simulink model "PrmM_CustomerLimits"  (R2018b)
settings: Solver=FixedStepDiscrete  StartTime=0.0  StopTime=20  RelTol=1e-3  EnableMultiTasking=on
undefined symbols (not defined in the file): CS_PrmM_nHSpdBd_XDF32, CS_PrmM_nLwrSpdBd_XDF32, CS_PrmM_uDcMaxVoltMode_XDF32, CS_PrmM_uDcMinVoltMode_XDF32
libraries: CalibrationLib x1
(part 2 of 2)

== stateflow chart PrmM_CustomerLimits/Test Sequence ==
  settings: updateMethod=DISCRETE  sampleTime=0.001  stateMachineType=SIMPLIFIED_MACHINE
  state Run
    %% Initialize data outputs.
    DrvM_Inp_sState = AD_DrvM_tSTATEIDX_E.CS_DrvM_STATE_Idle;
    ModeReqInt_Inp_sIntReqMode = AD_DrvM_tSTATEIDX_E.CS_DrvM_STATE_Idle;
    VoltLimExt_Inp_uReqdMinBattU = single(0);
    TqReqLim_Inp_mTqMax = single(0);
    VoltLimExt_Inp_uReqdMaxBattU = single(0);
    PwrLimExt_Inp_pPwrMinLim = single(0);
    PwrLimExt_Inp_pPwrMaxLim = single(0);
    TqDesGrdtExt_Inp_TqDesGrdtExt = single(0);
    Rotp_Inp_nSpdMecl = single(0);
    CurrLimExt_Inp_iReqdMinBattI = single(0);
    ExtTarTqReq_Inp_mReqTqEM = single(0);
    TqLimExt_Inp_mTqLimMin = single(0);
    CurrLimExt_Inp_iReqdMaxBattI = single(0);
    TqLimExt_Inp_mTqLimMax = single(0);
    ExtTarTqReq_Inp_nReqdSpdEM = single(0);
    ExtTarTqReq_Inp_uReqUEM = single(0);
    TqReqLim_Inp_mTqMin = single(0);
    ActTq_Inp_mDragTq = single(0);
    IDcLim_Inp_IDcLimMinInt=single(-290);
    IDcLim_Inp_IDcLimMaxInt=single(360);
    SplyU48_uU48=single(48);
    ElmTqLim_mTqMin=single(-70);
  state TorqueLimits
    state SpeedMode
      DrvM_Inp_sState = AD_DrvM_tSTATEIDX_E.CS_DrvM_STATE_Spd;
      state ExternalLimitsAreTheStrictest
        TqLimExt_Inp_mTqLimMax=single(20);
        TqLimExt_Inp_mTqLimMin=single(-20);
        TqReqLim_Inp_mTqMax=single(65);
        TqReqLim_Inp_mTqMin=single(-60);
        state wait
        state verfiy
          verify(abs(TqLimTarTqCtrl_Outp_mTqLimMax-TqLimExt_Inp_mTqLimMax)<Tolerance)
          verify(abs(TqLimTarTqCtrl_Outp_mTqLimMin-TqLimExt_Inp_mTqLimMin)<Tolerance)
          verify(abs(PwrLimExtCust_Outp_pPwrMaxLim-PwrLimExt_Inp_pPwrMaxLim)<Tolerance)
          verify(abs(PwrLimExtCust_Outp_pPwrMinLim-PwrLimExt_Inp_pPwrMinLim)<Tolerance)
        (default) -> TorqueLimits.SpeedMode.ExternalLimitsAreTheStrictest.wait
        TorqueLimits.SpeedMode.ExternalLimitsAreTheStrictest.wait -> TorqueLimits.SpeedMode.ExternalLimitsAreTheStrictest.verfiy : [after(0.1,sec)
            | ]
      state DeratingLimitsAreTheStrictest
        TqLimExt_Inp_mTqLimMax=single(65);
        TqLimExt_Inp_mTqLimMin=single(-65);
        TqReqLim_Inp_mTqMax=single(20);
        TqReqLim_Inp_mTqMin=single(-20);
        state wait
        state verfiy
          verify(abs(TqLimTarTqCtrl_Outp_mTqLimMax-TqReqLim_Inp_mTqMax)<Tolerance)
          verify(abs(TqLimTarTqCtrl_Outp_mTqLimMin-TqReqLim_Inp_mTqMin)<Tolerance)
          verify(abs(PwrLimExtCust_Outp_pPwrMaxLim-PwrLimExt_Inp_pPwrMaxLim)<Tolerance)
          verify(abs(PwrLimExtCust_Outp_pPwrMinLim-PwrLimExt_Inp_pPwrMinLim)<Tolerance)
        (default) -> TorqueLimits.SpeedMode.DeratingLimitsAreTheStrictest.wait
        TorqueLimits.SpeedMode.DeratingLimitsAreTheStrictest.wait -> TorqueLimits.SpeedMode.DeratingLimitsAreTheStrictest.verfiy : [after(0.1,sec)
            | ]
      state ExtLimitsAboveIntLimits
        TqLimExt_Inp_mTqLimMax=single(65);
        TqLimExt_Inp_mTqLimMin=single(50);
        TqReqLim_Inp_mTqMax=single(20);
        TqReqLim_Inp_mTqMin=single(-65);
        state wait
        state verfiy
          verify(abs(TqLimTarTqCtrl_Outp_mTqLimMax-TqReqLim_Inp_mTqMax)<Tolerance)
          verify(abs(TqLimTarTqCtrl_Outp_mTqLimMin-TqReqLim_Inp_mTqMin)<Tolerance)
          verify(abs(PwrLimExtCust_Outp_pPwrMaxLim-PwrLimExt_Inp_pPwrMaxLim)<Tolerance)
          verify(abs(PwrLimExtCust_Outp_pPwrMinLim-PwrLimExt_Inp_pPwrMinLim)<Tolerance)
        (default) -> TorqueLimits.SpeedMode.ExtLimitsAboveIntLimits.wait
        TorqueLimits.SpeedMode.ExtLimitsAboveIntLimits.wait -> TorqueLimits.SpeedMode.ExtLimitsAboveIntLimits.verfiy : [after(0.1,sec)
            | ]
      state ExtLimitsBelowIntLimits
        TqLimExt_Inp_mTqLimMax=single(-20);
        TqLimExt_Inp_mTqLimMin=single(-65);
        TqReqLim_Inp_mTqMax=single(65);
        TqReqLim_Inp_mTqMin=single(20);
        state wait
        state verfiy
          verify(abs(TqLimTarTqCtrl_Outp_mTqLimMax-TqReqLim_Inp_mTqMax)<Tolerance)
          verify(abs(TqLimTarTqCtrl_Outp_mTqLimMin-TqReqLim_Inp_mTqMin)<Tolerance)
          verify(abs(PwrLimExtCust_Outp_pPwrMaxLim-PwrLimExt_Inp_pPwrMaxLim)<Tolerance)
          verify(abs(PwrLimExtCust_Outp_pPwrMinLim-PwrLimExt_Inp_pPwrMinLim)<Tolerance)
        (default) -> TorqueLimits.SpeedMode.ExtLimitsBelowIntLimits.wait
        TorqueLimits.SpeedMode.ExtLimitsBelowIntLimits.wait -> TorqueLimits.SpeedMode.ExtLimitsBelowIntLimits.verfiy : [after(0.1,sec)
            | ]
      state InvalidExternalTorqueLimits
        TqLimExt_Inp_mTqLimMax=single(-20);
        TqLimExt_Inp_mTqLimMin=single(20);
        TqReqLim_Inp_mTqMax=single(20);
        TqReqLim_Inp_mTqMin=single(-20);
        state wait
        state verfiy
          verify(abs(TqLimTarTqCtrl_Outp_mTqLimMax-TqReqLim_Inp_mTqMax)<Tolerance)
          verify(abs(TqLimTarTqCtrl_Outp_mTqLimMin-TqReqLim_Inp_mTqMin)<Tolerance)
          verify(abs(PwrLimExtCust_Outp_pPwrMaxLim-PwrLimExt_Inp_pPwrMaxLim)<Tolerance)
          verify(abs(PwrLimExtCust_Outp_pPwrMinLim-PwrLimExt_Inp_pPwrMinLim)<Tolerance)
        (default) -> TorqueLimits.SpeedMode.InvalidExternalTorqueLimits.wait
        TorqueLimits.SpeedMode.InvalidExternalTorqueLimits.wait -> TorqueLimits.SpeedMode.InvalidExternalTorqueLimits.verfiy : [after(0.1,sec)
            | ]
      state InvalidInternalTorqueLimits
        TqLimExt_Inp_mTqLimMax=single(-20);
        TqLimExt_Inp_mTqLimMin=single(20);
        TqReqLim_Inp_mTqMax=single(-20);
        TqReqLim_Inp_mTqMin=single(20);
        state wait
        state verfiy
          verify(abs(TqLimTarTqCtrl_Outp_mTqLimMax-TqReqLim_Inp_mTqMin)<Tolerance)
          verify(abs(TqLimTarTqCtrl_Outp_mTqLimMin-TqReqLim_Inp_mTqMax)<Tolerance)
          verify(abs(PwrLimExtCust_Outp_pPwrMaxLim-PwrLimExt_Inp_pPwrMaxLim)<Tolerance)
          verify(abs(PwrLimExtCust_Outp_pPwrMinLim-PwrLimExt_Inp_pPwrMinLim)<Tolerance)
        (default) -> TorqueLimits.SpeedMode.InvalidInternalTorqueLimits.wait
        TorqueLimits.SpeedMode.InvalidInternalTorqueLimits.wait -> TorqueLimits.SpeedMode.InvalidInternalTorqueLimits.verfiy : [after(0.1,sec)
            | ]
      (default) -> TorqueLimits.SpeedMode.ExternalLimitsAreTheStrictest
      TorqueLimits.SpeedMode.ExternalLimitsAreTheStrictest -> TorqueLimits.SpeedMode.DeratingLimitsAreTheStrictest : [after(0.5,sec)
          | ]
      TorqueLimits.SpeedMode.DeratingLimitsAreTheStrictest -> TorqueLimits.SpeedMode.ExtLimitsAboveIntLimits : [after(0.5,sec)
          | ]
      TorqueLimits.SpeedMode.ExtLimitsAboveIntLimits -> TorqueLimits.SpeedMode.ExtLimitsBelowIntLimits : [after(0.5,sec)
          | ]
      TorqueLimits.SpeedMode.ExtLimitsBelowIntLimits -> InvalidExternalTorqueLimits : [after(0.5,sec)
          | ]
      InvalidExternalTorqueLimits -> InvalidInternalTorqueLimits : [after(0.5,sec)
          | ]
    state TorqueMode
      DrvM_Inp_sState = AD_DrvM_tSTATEIDX_E.CS_DrvM_STATE_Tq;
      TqLimExt_Inp_mTqLimMax=single(65);
      TqLimExt_Inp_mTqLimMin=single(-65);
      TqReqLim_Inp_mTqMax=single(20);
      TqReqLim_Inp_mTqMin=single(-20);
      state wait
      state verfiy
        verify(abs(TqLimTarTqCtrl_Outp_mTqLimMax-TqLimExt_Inp_mTqLimMax)<Tolerance)
        verify(abs(TqLimTarTqCtrl_Outp_mTqLimMin-TqLimExt_Inp_mTqLimMin)<Tolerance)
        verify(abs(PwrLimExtCust_Outp_pPwrMaxLim-PwrLimExt_Inp_pPwrMaxLim)<Tolerance)
        verify(abs(PwrLimExtCust_Outp_pPwrMinLim-PwrLimExt_Inp_pPwrMinLim)<Tolerance)
      (default) -> TorqueLimits.TorqueMode.wait
      TorqueLimits.TorqueMode.wait -> TorqueLimits.TorqueMode.verfiy : [after(0.1,sec)
          | ]
    state VoltageMode
      DrvM_Inp_sState = AD_DrvM_tSTATEIDX_E.CS_DrvM_STATE_Volt;
      state MaximumTorqueHigherThanDragTorque
        TqLimExt_Inp_mTqLimMax=single(65);
        TqLimExt_Inp_mTqLimMin=single(-65);
        TqReqLim_Inp_mTqMax=single(20);
        TqReqLim_Inp_mTqMin=single(-20);
        ActTq_Inp_mDragTq=single(0.3);
        ElmTqLim_mTqMin=single(-20);
        state wait
        state verfiy
          verify(abs(TqLimTarTqCtrl_Outp_mTqLimMax+ActTq_Inp_mDragTq)<Tolerance)
          verify(abs(TqLimTarTqCtrl_Outp_mTqLimMin+ActTq_Inp_mDragTq)<Tolerance)
          verify(abs(PwrLimExtCust_Outp_pPwrMaxLim-PwrLimExt_Inp_pPwrMaxLim)<Tolerance)
          verify(abs(PwrLimExtCust_Outp_pPwrMinLim-PwrLimExt_Inp_pPwrMinLim)<Tolerance)
        (default) -> TorqueLimits.VoltageMode.MaximumTorqueHigherThanDragTorque.wait
        TorqueLimits.VoltageMode.MaximumTorqueHigherThanDragTorque.wait -> TorqueLimits.VoltageMode.MaximumTorqueHigherThanDragTorque.verfiy : [after(0.1,sec)
            | ]
      state SpeedHigherThanHSpdBd
        %TqReqLim_Inp_mTqMax=single(0);
        Rotp_Inp_nSpdMecl=single(0.99+CS_PrmM_nHSpdBd_XDF32);
        state wait
        state verfiy
          verify(abs(TqLimTarTqCtrl_Outp_mTqLimMax+ActTq_Inp_mDragTq)<Tolerance)
          verify(abs(TqLimTarTqCtrl_Outp_mTqLimMin-ElmTqLim_mTqMin)<Tolerance)
          verify(abs(PwrLimExtCust_Outp_pPwrMaxLim-PwrLimExt_Inp_pPwrMaxLim)<Tolerance)
          verify(abs(PwrLimExtCust_Outp_pPwrMinLim-PwrLimExt_Inp_pPwrMinLim)<Tolerance)
        (default) -> TorqueLimits.VoltageMode.SpeedHigherThanHSpdBd.wait
        TorqueLimits.VoltageMode.SpeedHigherThanHSpdBd.wait -> TorqueLimits.VoltageMode.SpeedHigherThanHSpdBd.verfiy : [after(0.1,sec)
            | ]
      (default) -> TorqueLimits.VoltageMode.MaximumTorqueHigherThanDragTorque
      TorqueLimits.VoltageMode.MaximumTorqueHigherThanDragTorque -> SpeedHigherThanHSpdBd : [after(0.5,sec)
          | ]
    state CommuincationlossMode
      DrvM_Inp_sState = AD_DrvM_tSTATEIDX_E.CS_DrvM_STATE_ComLoss
      state MaximumTorqueHigherThanDragTorque
        TqLimExt_Inp_mTqLimMax=single(65);
        TqLimExt_Inp_mTqLimMin=single(-65);
        TqReqLim_Inp_mTqMax=single(20);
        TqReqLim_Inp_mTqMin=single(-20);
        Rotp_Inp_nSpdMecl=single(-500);
        ActTq_Inp_mDragTq=single(-0.3);
        state wait
        state verfiy
          verify(abs(TqLimTarTqCtrl_Outp_mTqLimMax+ActTq_Inp_mDragTq)<Tolerance)
          verify(abs(TqLimTarTqCtrl_Outp_mTqLimMin+ActTq_Inp_mDragTq)<Tolerance)
          verify(abs(PwrLimExtCust_Outp_pPwrMaxLim-PwrLimExt_Inp_pPwrMaxLim)<Tolerance)
          verify(abs(PwrLimExtCust_Outp_pPwrMinLim-PwrLimExt_Inp_pPwrMinLim)<Tolerance)
        (default) -> TorqueLimits.CommuincationlossMode.MaximumTorqueHigherThanDragTorque.wait
        TorqueLimits.CommuincationlossMode.MaximumTorqueHigherThanDragTorque.wait -> TorqueLimits.CommuincationlossMode.MaximumTorqueHigherThanDragTorque.verfiy : [after(0.1,sec)
            | ]
      state SpeedBtwHSpdBdAndLwrSpdBd
        %TqReqLim_Inp_mTqMax=single(0);
        Rotp_Inp_nSpdMecl=CS_PrmM_nLwrSpdBd_XDF32+single(50);
        ActTq_Inp_mDragTq=single(0.3);
        TqMinInterpol=(ElmTqLim_mTqMin+ActTq_Inp_mDragTq)*(Rotp_Inp_nSpdMecl-CS_PrmM_nLwrSpdBd_XDF32)/...
        (CS_PrmM_nHSpdBd_XDF32-CS_PrmM_nLwrSpdBd_XDF32)-ActTq_Inp_mDragTq;
        state wait
        state verfiy
          verify(abs(TqLimTarTqCtrl_Outp_mTqLimMax+ActTq_Inp_mDragTq)<Tolerance)
          verify(abs(TqLimTarTqCtrl_Outp_mTqLimMin-TqMinInterpol)<Tolerance)
          verify(abs(PwrLimExtCust_Outp_pPwrMaxLim-PwrLimExt_Inp_pPwrMaxLim)<Tolerance)
          verify(abs(PwrLimExtCust_Outp_pPwrMinLim-PwrLimExt_Inp_pPwrMinLim)<Tolerance)
        (default) -> TorqueLimits.CommuincationlossMode.SpeedBtwHSpdBdAndLwrSpdBd.wait
        TorqueLimits.CommuincationlossMode.SpeedBtwHSpdBdAndLwrSpdBd.wait -> TorqueLimits.CommuincationlossMode.SpeedBtwHSpdBdAndLwrSpdBd.verfiy : [after(0.1,sec)
            | ]
      (default) -> TorqueLimits.CommuincationlossMode.MaximumTorqueHigherThanDragTorque
      TorqueLimits.CommuincationlossMode.MaximumTorqueHigherThanDragTorque -> SpeedBtwHSpdBdAndLwrSpdBd : [after(0.5,sec)
          | ]
    state BatteryDisconnectedMode
      DrvM_Inp_sState = AD_DrvM_tSTATEIDX_E.CS_DrvM_STATE_BattDiscnctd;
      state MaximumTorqueHigherThanDargTorque
        TqLimExt_Inp_mTqLimMax=single(65);
        TqLimExt_Inp_mTqLimMin=single(-65);
        TqReqLim_Inp_mTqMax=single(20);
        TqReqLim_Inp_mTqMin=single(-20);
        ActTq_Inp_mDragTq=single(0.3);
        state wait
        state verfiy
          verify(abs(TqLimTarTqCtrl_Outp_mTqLimMax+ActTq_Inp_mDragTq)<Tolerance)
          verify(abs(TqLimTarTqCtrl_Outp_mTqLimMin-TqReqLim_Inp_mTqMin)<Tolerance)
          verify(abs(PwrLimExtCust_Outp_pPwrMaxLim-PwrLimExt_Inp_pPwrMaxLim)<Tolerance)
          verify(abs(PwrLimExtCust_Outp_pPwrMinLim-PwrLimExt_Inp_pPwrMinLim)<Tolerance)
        (default) -> TorqueLimits.BatteryDisconnectedMode.MaximumTorqueHigherThanDargTorque.wait
        TorqueLimits.BatteryDisconnectedMode.MaximumTorqueHigherThanDargTorque.wait -> TorqueLimits.BatteryDisconnectedMode.MaximumTorqueHigherThanDargTorque.verfiy : [after(0.1,sec)
            | ]
      state MaximumTorqueLowerThanDargTorque
        TqLimExt_Inp_mTqLimMax=single(0);
        ActTq_Inp_mDragTq=single(-0.3);
        Rotp_Inp_nSpdMecl=single(-500);
        state wait
        state verfiy
          verify(abs(TqLimTarTqCtrl_Outp_mTqLimMax-TqLimExt_Inp_mTqLimMax)<Tolerance)
          verify(abs(TqLimTarTqCtrl_Outp_mTqLimMin-TqReqLim_Inp_mTqMin)<Tolerance)
          verify(abs(PwrLimExtCust_Outp_pPwrMaxLim-PwrLimExt_Inp_pPwrMaxLim)<Tolerance)
          verify(abs(PwrLimExtCust_Outp_pPwrMinLim-PwrLimExt_Inp_pPwrMinLim)<Tolerance)
        (default) -> TorqueLimits.BatteryDisconnectedMode.MaximumTorqueLowerThanDargTorque.wait
        TorqueLimits.BatteryDisconnectedMode.MaximumTorqueLowerThanDargTorque.wait -> TorqueLimits.BatteryDisconnectedMode.MaximumTorqueLowerThanDargTorque.verfiy : [after(0.1,sec)
            | ]
      (default) -> MaximumTorqueHigherThanDargTorque
      MaximumTorqueHigherThanDargTorque -> MaximumTorqueLowerThanDargTorque : [after(0.5,sec)
          | ]
    (default) -> SpeedMode
    SpeedMode -> TorqueMode : [after(3.5,sec)
        | ]
    TorqueMode -> VoltageMode : [after(0.5,sec)
        | ]
    VoltageMode -> CommuincationlossMode : [after(1,sec)
        | ]
    CommuincationlossMode -> BatteryDisconnectedMode : [after(1,sec)
        | ]
  state TorqueGrandient
    state InternalLimitsAreSelected
      state wait
      state verfiy
        verify(abs(PrmM_Outp_mMaxTqGrdtInt-single(1000))<Tolerance)
        verify(abs(PwrLimExtCust_Outp_pPwrMaxLim-PwrLimExt_Inp_pPwrMaxLim)<Tolerance)
        verify(abs(PwrLimExtCust_Outp_pPwrMinLim-PwrLimExt_Inp_pPwrMinLim)<Tolerance)
      (default) -> TorqueGrandient.InternalLimitsAreSelected.wait
      TorqueGrandient.InternalLimitsAreSelected.wait -> TorqueGrandient.InternalLimitsAreSelected.verfiy : [(CS_PrmM_fTqGrdSelect_XDB==true)&&after(0.1,sec)
          | ]
    state ExternalLimitsAreSelected
      state ExternalTorqueGrandientIsHigherThan2000Nm
        TqDesGrdtExt_Inp_TqDesGrdtExt = single(2500);
        state wait
        state verfiy
          verify(abs(PrmM_Outp_mMaxTqGrdtInt-single(2000))<Tolerance)
          verify(abs(PwrLimExtCust_Outp_pPwrMaxLim-PwrLimExt_Inp_pPwrMaxLim)<Tolerance)
          verify(abs(PwrLimExtCust_Outp_pPwrMinLim-PwrLimExt_Inp_pPwrMinLim)<Tolerance)
        (default) -> TorqueGrandient.ExternalLimitsAreSelected.ExternalTorqueGrandientIsHigherThan2000Nm.wait
        TorqueGrandient.ExternalLimitsAreSelected.ExternalTorqueGrandientIsHigherThan2000Nm.wait -> TorqueGrandient.ExternalLimitsAreSelected.ExternalTorqueGrandientIsHigherThan2000Nm.verfiy : [after(0.1,sec)
            | ]
      state ExternalTorqueGrandientIsLowerThan2000Nm
        TqDesGrdtExt_Inp_TqDesGrdtExt = single(1500);
        state wait
        state verfiy
          verify(abs(PrmM_Outp_mMaxTqGrdtInt-TqDesGrdtExt_Inp_TqDesGrdtExt)<Tolerance)
          verify(abs(PwrLimExtCust_Outp_pPwrMaxLim-PwrLimExt_Inp_pPwrMaxLim)<Tolerance)
          verify(abs(PwrLimExtCust_Outp_pPwrMinLim-PwrLimExt_Inp_pPwrMinLim)<Tolerance)
        (default) -> TorqueGrandient.ExternalLimitsAreSelected.ExternalTorqueGrandientIsLowerThan2000Nm.wait
        TorqueGrandient.ExternalLimitsAreSelected.ExternalTorqueGrandientIsLowerThan2000Nm.wait -> TorqueGrandient.ExternalLimitsAreSelected.ExternalTorqueGrandientIsLowerThan2000Nm.verfiy : [after(0.1,sec)
            | ]
      state ExternalTorqueGrandientIs0Nm
        TqDesGrdtExt_Inp_TqDesGrdtExt = single(0);
        state wait
        state verfiy
          verify(abs(PrmM_Outp_mMaxTqGrdtInt-single(1000))<Tolerance)
          verify(abs(PwrLimExtCust_Outp_pPwrMaxLim-PwrLimExt_Inp_pPwrMaxLim)<Tolerance)
          verify(abs(PwrLimExtCust_Outp_pPwrMinLim-PwrLimExt_Inp_pPwrMinLim)<Tolerance)
        (default) -> TorqueGrandient.ExternalLimitsAreSelected.ExternalTorqueGrandientIs0Nm.wait
        TorqueGrandient.ExternalLimitsAreSelected.ExternalTorqueGrandientIs0Nm.wait -> TorqueGrandient.ExternalLimitsAreSelected.ExternalTorqueGrandientIs0Nm.verfiy : [after(0.1,sec)
            | ]
      (default) -> ExternalTorqueGrandientIsHigherThan2000Nm
      ExternalTorqueGrandientIsHigherThan2000Nm -> ExternalTorqueGrandientIsLowerThan2000Nm : [after(0.5,sec)
          | ]
      ExternalTorqueGrandientIsLowerThan2000Nm -> ExternalTorqueGrandientIs0Nm : [after(0.5,sec)
          | ]
    (default) -> InternalLimitsAreSelected
    InternalLimitsAreSelected -> ExternalLimitsAreSelected : [CS_PrmM_fTqGrdSelect_XDB==false
        | ]
  state VoltageLimits
    DrvM_Inp_sState = AD_DrvM_tSTATEIDX_E.CS_DrvM_STATE_Volt;
    state ExternalLimitsAreTheStrictest
      if CS_PrmM_fTqGrdSelect_XDB
      VoltLimExt_Inp_uReqdMaxBattU=single(CS_PrmM_uDcMaxVoltMode_XDF32-5);
      VoltLimExt_Inp_uReqdMinBattU=single(CS_PrmM_uDcMinVoltMode_XDF32+5);
      else
      VoltLimExt_Inp_uReqdMaxBattU=single(CS_PrmM_uDcMinVoltMode_XDF32-5);
      VoltLimExt_Inp_uReqdMinBattU=single(CS_PrmM_uDcMaxVoltMode_XDF32+5);
      end
      state wait
      state verfiy
        verify(abs(VoltLimExtCust_Outp_uReqdMaxBattU-VoltLimExt_Inp_uReqdMaxBattU)<Tolerance)
        verify(abs(VoltLimExtCust_Outp_uReqdMinBattU-VoltLimExt_Inp_uReqdMinBattU)<Tolerance)
        verify(abs(PwrLimExtCust_Outp_pPwrMaxLim-PwrLimExt_Inp_pPwrMaxLim)<Tolerance)
        verify(abs(PwrLimExtCust_Outp_pPwrMinLim-PwrLimExt_Inp_pPwrMinLim)<Tolerance)
      (default) -> VoltageLimits.ExternalLimitsAreTheStrictest.wait
      VoltageLimits.ExternalLimitsAreTheStrictest.wait -> VoltageLimits.ExternalLimitsAreTheStrictest.verfiy : [after(0.1,sec)
          | ]
    state DeratingLimitsAreTheStrictest
      if CS_PrmM_fTqGrdSelect_XDB
      VoltLimExt_Inp_uReqdMaxBattU=single(CS_PrmM_uDcMaxVoltMode_XDF32+5);
      VoltLimExt_Inp_uReqdMinBattU=single(CS_PrmM_uDcMinVoltMode_XDF32-5);
      else
      VoltLimExt_Inp_uReqdMaxBattU=single(CS_PrmM_uDcMinVoltMode_XDF32+5);
      VoltLimExt_Inp_uReqdMinBattU=single(CS_PrmM_uDcMaxVoltMode_XDF32-5);
      end
      state wait
      state verfiy
        if ~CS_PrmM_fTqGrdSelect_XDB
        verify(abs(VoltLimExtCust_Outp_uReqdMaxBattU-PrmM_Outp_uDcMinAllwd)<Tolerance)
        verify(abs(VoltLimExtCust_Outp_uReqdMinBattU-PrmM_Outp_uDcMaxAllwd)<Tolerance)
        else
        verify(abs(VoltLimExtCust_Outp_uReqdMaxBattU-PrmM_Outp_uDcMaxAllwd)<Tolerance)
        verify(abs(VoltLimExtCust_Outp_uReqdMinBattU-PrmM_Outp_uDcMinAllwd)<Tolerance)
        end
        verify(abs(PwrLimExtCust_Outp_pPwrMaxLim-PwrLimExt_Inp_pPwrMaxLim)<Tolerance)
        verify(abs(PwrLimExtCust_Outp_pPwrMinLim-PwrLimExt_Inp_pPwrMinLim)<Tolerance)
      (default) -> VoltageLimits.DeratingLimitsAreTheStrictest.wait
      VoltageLimits.DeratingLimitsAreTheStrictest.wait -> VoltageLimits.DeratingLimitsAreTheStrictest.verfiy : [after(0.1,sec)
          | ]
    state ExtLimitsAboveIntLimits
      if CS_PrmM_fTqGrdSelect_XDB
      VoltLimExt_Inp_uReqdMaxBattU=single(2*CS_PrmM_uDcMaxVoltMode_XDF32);
      VoltLimExt_Inp_uReqdMinBattU=single(CS_PrmM_uDcMaxVoltMode_XDF32 +5);
      else
      VoltLimExt_Inp_uReqdMaxBattU=single(2*CS_PrmM_uDcMinVoltMode_XDF32);
      VoltLimExt_Inp_uReqdMinBattU=single(CS_PrmM_uDcMinVoltMode_XDF32+5);
      end
      state wait
      state verfiy
        if ~CS_PrmM_fTqGrdSelect_XDB
        verify(abs(VoltLimExtCust_Outp_uReqdMaxBattU-PrmM_Outp_uDcMinAllwd)<Tolerance)
        verify(abs(VoltLimExtCust_Outp_uReqdMinBattU-PrmM_Outp_uDcMaxAllwd)<Tolerance)
        else
        verify(abs(VoltLimExtCust_Outp_uReqdMaxBattU-PrmM_Outp_uDcMaxAllwd)<Tolerance)
        verify(abs(VoltLimExtCust_Outp_uReqdMinBattU-PrmM_Outp_uDcMinAllwd)<Tolerance)
        end
        verify(abs(PwrLimExtCust_Outp_pPwrMaxLim-PwrLimExt_Inp_pPwrMaxLim)<Tolerance)
        verify(abs(PwrLimExtCust_Outp_pPwrMinLim-PwrLimExt_Inp_pPwrMinLim)<Tolerance)
      (default) -> VoltageLimits.ExtLimitsAboveIntLimits.wait
      VoltageLimits.ExtLimitsAboveIntLimits.wait -> VoltageLimits.ExtLimitsAboveIntLimits.verfiy : [after(0.1,sec)
          | ]
    state ExtLimitsBelowIntLimits
      if CS_PrmM_fTqGrdSelect_XDB
      VoltLimExt_Inp_uReqdMaxBattU=single(CS_PrmM_uDcMinVoltMode_XDF32-5);
      VoltLimExt_Inp_uReqdMinBattU=single(CS_PrmM_uDcMinVoltMode_XDF32/2);
      else
      VoltLimExt_Inp_uReqdMaxBattU=single(CS_PrmM_uDcMaxVoltMode_XDF32-5);
      VoltLimExt_Inp_uReqdMinBattU=single(CS_PrmM_uDcMaxVoltMode_XDF32/2);
      end
      state wait
      state verfiy
        if ~CS_PrmM_fTqGrdSelect_XDB
        verify(abs(VoltLimExtCust_Outp_uReqdMaxBattU-PrmM_Outp_uDcMinAllwd)<Tolerance)
        verify(abs(VoltLimExtCust_Outp_uReqdMinBattU-PrmM_Outp_uDcMaxAllwd)<Tolerance)
        else
        verify(abs(VoltLimExtCust_Outp_uReqdMaxBattU-PrmM_Outp_uDcMaxAllwd)<Tolerance)
        verify(abs(VoltLimExtCust_Outp_uReqdMinBattU-PrmM_Outp_uDcMinAllwd)<Tolerance)
        end
        verify(abs(PwrLimExtCust_Outp_pPwrMaxLim-PwrLimExt_Inp_pPwrMaxLim)<Tolerance)
        verify(abs(PwrLimExtCust_Outp_pPwrMinLim-PwrLimExt_Inp_pPwrMinLim)<Tolerance)
      (default) -> VoltageLimits.ExtLimitsBelowIntLimits.wait
      VoltageLimits.ExtLimitsBelowIntLimits.wait -> VoltageLimits.ExtLimitsBelowIntLimits.verfiy : [after(0.1,sec)
          | ]
    state InvalidExternalVoltageLimits
      VoltLimExt_Inp_uReqdMaxBattU=single(22);
      VoltLimExt_Inp_uReqdMinBattU=single(40);
      state wait
      state verfiy
        if ~CS_PrmM_fTqGrdSelect_XDB
        verify(abs(VoltLimExtCust_Outp_uReqdMaxBattU-PrmM_Outp_uDcMinAllwd)<Tolerance)
        verify(abs(VoltLimExtCust_Outp_uReqdMinBattU-PrmM_Outp_uDcMaxAllwd)<Tolerance)
        else
        verify(abs(VoltLimExtCust_Outp_uReqdMaxBattU-PrmM_Outp_uDcMaxAllwd)<Tolerance)
        verify(abs(VoltLimExtCust_Outp_uReqdMinBattU-PrmM_Outp_uDcMinAllwd)<Tolerance)
        end
        verify(abs(PwrLimExtCust_Outp_pPwrMaxLim-PwrLimExt_Inp_pPwrMaxLim)<Tolerance)
        verify(abs(PwrLimExtCust_Outp_pPwrMinLim-PwrLimExt_Inp_pPwrMinLim)<Tolerance)
      (default) -> VoltageLimits.InvalidExternalVoltageLimits.wait
      VoltageLimits.InvalidExternalVoltageLimits.wait -> VoltageLimits.InvalidExternalVoltageLimits.verfiy : [after(0.1,sec)
          | ]
    (default) -> VoltageLimits.ExternalLimitsAreTheStrictest
    VoltageLimits.ExternalLimitsAreTheStrictest -> VoltageLimits.DeratingLimitsAreTheStrictest : [after(0.5,sec)
        | ]
    VoltageLimits.DeratingLimitsAreTheStrictest -> VoltageLimits.ExtLimitsAboveIntLimits : [after(0.5,sec)
        | ]
    VoltageLimits.ExtLimitsAboveIntLimits -> VoltageLimits.ExtLimitsBelowIntLimits : [after(0.5,sec)
        | ]
    VoltageLimits.ExtLimitsBelowIntLimits -> InvalidExternalVoltageLimits : [after(0.5,sec)
        | ]
  state CurrentLimits
    state ExternalLimitsAreTheStrictest
      CurrLimExt_Inp_iReqdMaxBattI=single(300);
      CurrLimExt_Inp_iReqdMinBattI =single(-200);
      IDcLim_Inp_IDcLimMinInt=single(-290);
      IDcLim_Inp_IDcLimMaxInt=single(360);
      state wait
      state verfiy
        verify(abs(CurrLimExtCust_Outp_iReqdMaxBattI-CurrLimExt_Inp_iReqdMaxBattI)<Tolerance)
        verify(abs(CurrLimExtCust_Outp_iReqdMinBattI-CurrLimExt_Inp_iReqdMinBattI)<Tolerance)
        verify(abs(PwrLimExtCust_Outp_pPwrMaxLim-PwrLimExt_Inp_pPwrMaxLim)<Tolerance)
        verify(abs(PwrLimExtCust_Outp_pPwrMinLim-PwrLimExt_Inp_pPwrMinLim)<Tolerance)
      (default) -> CurrentLimits.ExternalLimitsAreTheStrictest.wait
      CurrentLimits.ExternalLimitsAreTheStrictest.wait -> CurrentLimits.ExternalLimitsAreTheStrictest.verfiy : [after(0.1,sec)
          | ]
    state DeratingLimitsAreTheStrictest
      CurrLimExt_Inp_iReqdMaxBattI=single(400);
      CurrLimExt_Inp_iReqdMinBattI =single(-300);
      state wait
      state verfiy
        verify(abs(CurrLimExtCust_Outp_iReqdMaxBattI-IDcLim_Inp_IDcLimMaxInt)<Tolerance)
        verify(abs(CurrLimExtCust_Outp_iReqdMinBattI-IDcLim_Inp_IDcLimMinInt)<Tolerance)
        verify(abs(PwrLimExtCust_Outp_pPwrMaxLim-PwrLimExt_Inp_pPwrMaxLim)<Tolerance)
        verify(abs(PwrLimExtCust_Outp_pPwrMinLim-PwrLimExt_Inp_pPwrMinLim)<Tolerance)
      (default) -> CurrentLimits.DeratingLimitsAreTheStrictest.wait
      CurrentLimits.DeratingLimitsAreTheStrictest.wait -> CurrentLimits.DeratingLimitsAreTheStrictest.verfiy : [after(0.1,sec)
          | ]
    state ExtLimitsAboveIntLimits
      IDcLim_Inp_IDcLimMinInt=single(-290);
      IDcLim_Inp_IDcLimMaxInt=single(360);
      CurrLimExt_Inp_iReqdMaxBattI=single(2*IDcLim_Inp_IDcLimMaxInt);
      CurrLimExt_Inp_iReqdMinBattI =single(IDcLim_Inp_IDcLimMaxInt +5);
      state wait
      state verfiy
        verify(abs(CurrLimExtCust_Outp_iReqdMaxBattI-IDcLim_Inp_IDcLimMaxInt)<Tolerance)
        verify(abs(CurrLimExtCust_Outp_iReqdMinBattI-IDcLim_Inp_IDcLimMinInt)<Tolerance)
        verify(abs(PwrLimExtCust_Outp_pPwrMaxLim-PwrLimExt_Inp_pPwrMaxLim)<Tolerance)
        verify(abs(PwrLimExtCust_Outp_pPwrMinLim-PwrLimExt_Inp_pPwrMinLim)<Tolerance)
      (default) -> CurrentLimits.ExtLimitsAboveIntLimits.wait
      CurrentLimits.ExtLimitsAboveIntLimits.wait -> CurrentLimits.ExtLimitsAboveIntLimits.verfiy : [after(0.1,sec)
          | ]
    state ExtLimitsBelowIntLimits
      IDcLim_Inp_IDcLimMinInt=single(-290);
      IDcLim_Inp_IDcLimMaxInt=single(360);
      CurrLimExt_Inp_iReqdMaxBattI=single(IDcLim_Inp_IDcLimMinInt-5);
      CurrLimExt_Inp_iReqdMinBattI =single(2*IDcLim_Inp_IDcLimMinInt);
      state wait
      state verfiy
        verify(abs(CurrLimExtCust_Outp_iReqdMaxBattI-IDcLim_Inp_IDcLimMaxInt)<Tolerance)
        verify(abs(CurrLimExtCust_Outp_iReqdMinBattI-IDcLim_Inp_IDcLimMinInt)<Tolerance)
        verify(abs(PwrLimExtCust_Outp_pPwrMaxLim-PwrLimExt_Inp_pPwrMaxLim)<Tolerance)
        verify(abs(PwrLimExtCust_Outp_pPwrMinLim-PwrLimExt_Inp_pPwrMinLim)<Tolerance)
      (default) -> CurrentLimits.ExtLimitsBelowIntLimits.wait
      CurrentLimits.ExtLimitsBelowIntLimits.wait -> CurrentLimits.ExtLimitsBelowIntLimits.verfiy : [after(0.1,sec)
          | ]
    state InvalidExternalCurrentLimits
      CurrLimExt_Inp_iReqdMaxBattI=single(100);
      CurrLimExt_Inp_iReqdMinBattI =single(200);
      state wait
      state verfiy
        verify(abs(CurrLimExtCust_Outp_iReqdMaxBattI-IDcLim_Inp_IDcLimMaxInt)<Tolerance)
        verify(abs(CurrLimExtCust_Outp_iReqdMinBattI-IDcLim_Inp_IDcLimMinInt)<Tolerance)
      (default) -> CurrentLimits.InvalidExternalCurrentLimits.wait
      CurrentLimits.InvalidExternalCurrentLimits.wait -> CurrentLimits.InvalidExternalCurrentLimits.verfiy : [after(0.1,sec)
          | ]
    state InvalidInternalCurrentLimits
      CurrLimExt_Inp_iReqdMaxBattI=single(100);
      CurrLimExt_Inp_iReqdMinBattI =single(200);
      IDcLim_Inp_IDcLimMinInt=single(0);
      IDcLim_Inp_IDcLimMaxInt=single(-1);
      state wait
      state verfiy
        verify(abs(CurrLimExtCust_Outp_iReqdMaxBattI-IDcLim_Inp_IDcLimMinInt)<Tolerance)
        verify(abs(CurrLimExtCust_Outp_iReqdMinBattI-IDcLim_Inp_IDcLimMaxInt)<Tolerance)
        verify(abs(PwrLimExtCust_Outp_pPwrMaxLim-PwrLimExt_Inp_pPwrMaxLim)<Tolerance)
        verify(abs(PwrLimExtCust_Outp_pPwrMinLim-PwrLimExt_Inp_pPwrMinLim)<Tolerance)
      (default) -> CurrentLimits.InvalidInternalCurrentLimits.wait
      CurrentLimits.InvalidInternalCurrentLimits.wait -> CurrentLimits.InvalidInternalCurrentLimits.verfiy : [after(0.1,sec)
          | ]
    (default) -> CurrentLimits.ExternalLimitsAreTheStrictest
    CurrentLimits.ExternalLimitsAreTheStrictest -> CurrentLimits.DeratingLimitsAreTheStrictest : [after(0.5,sec)
        | ]
    CurrentLimits.DeratingLimitsAreTheStrictest -> CurrentLimits.ExtLimitsAboveIntLimits : [after(0.5,sec)
        | ]
    CurrentLimits.ExtLimitsAboveIntLimits -> CurrentLimits.ExtLimitsBelowIntLimits : [after(0.5,sec)
        | ]
    CurrentLimits.ExtLimitsBelowIntLimits -> InvalidExternalCurrentLimits : [after(0.5,sec)
        | ]
    InvalidExternalCurrentLimits -> InvalidInternalCurrentLimits : [after(0.5,sec)
        | ]
  (default) -> Run
  Run -> TorqueLimits
  TorqueLimits -> TorqueGrandient : [after(7,sec)
      | ]
  TorqueGrandient -> VoltageLimits : [after(2,sec)
      | ]
  VoltageLimits -> CurrentLimits : [after(3,sec)
      | ]
  data: PrmM_Outp_uDcMinAllwd input AD_PrmM_tUDCMINALLWD size=[1]; PrmM_Outp_uDcMaxAllwd input AD_PrmM_tUDCMAXALLWD size=[1]; TqLimTarTqCtrl_Outp_mTqLimMax input AD_ComWrp_tMTQLIMMAX size=[1]; TqLimTarTqCtrl_Outp_mTqLimMin input AD_ComWrp_tMTQLIMMIN size=[1]; PrmM_Outp_mMaxTqGrdtInt input AD_PrmM_tMMAXTQGRDINT size=[1]; CurrLimExtCust_Outp_iReqdMinBattI input AD_ComWrp_tIREQDMINBATTI size=[1]; CurrLimExtCust_Outp_iReqdMaxBattI input AD_ComWrp_tIREQDMAXBATTI size=[1]; VoltLimExtCust_Outp_uReqdMinBattU input AD_ComWrp_tUREQDMINBATTU size=[1]; VoltLimExtCust_Outp_uReqdMaxBattU input AD_ComWrp_tUREQDMAXBATTU size=[1]; PwrLimExtCust_Outp_pPwrMinLim input; PwrLimExtCust_Outp_pPwrMaxLim input; DrvM_Inp_sState output Enum: AD_DrvM_tSTATEIDX_E size=[1]; ModeReqInt_Inp_sIntReqMode output Enum: AD_DrvM_tSTATEIDX_E size=[1]; ExtTarTqReq_Inp_mReqTqEM output AD_ComWrp_tMREQTQEM size=[1]; ExtTarTqReq_Inp_uReqUEM output AD_ComWrp_tUREQVOLTEM size=[1]; ExtTarTqReq_Inp_nReqdSpdEM output AD_ComWrp_tNREQDSPDEM size=[1]; TqReqLim_Inp_mTqMax output AD_TqReqLim_tMTQMAX size=[1]; TqReqLim_Inp_mTqMin output AD_TqReqLim_tMTQMIN size=[1]; TqLimExt_Inp_mTqLimMax output AD_ComWrp_tMTQLIMMAX size=[1]; TqLimExt_Inp_mTqLimMin output AD_ComWrp_tMTQLIMMIN size=[1]; VoltLimExt_Inp_uReqdMinBattU output AD_ComWrp_tUREQDMINBATTU size=[1]; VoltLimExt_Inp_uReqdMaxBattU output AD_ComWrp_tUREQDMAXBATTU size=[1]; CurrLimExt_Inp_iReqdMinBattI output AD_ComWrp_tIREQDMINBATTI size=[1]; CurrLimExt_Inp_iReqdMaxBattI output AD_ComWrp_tIREQDMAXBATTI size=[1]; PwrLimExt_Inp_pPwrMinLim output AD_ComWrp_tPPWRMINLIM size=[1]; PwrLimExt_Inp_pPwrMaxLim output AD_ComWrp_tPPWRMAXLIM size=[1]; TqDesGrdtExt_Inp_TqDesGrdtExt output size=[1]; Rotp_Inp_nSpdMecl output AD_RotP_tNSPDMECL size=[1]; IDcLim_Inp_IDcLimMinInt output; IDcLim_Inp_IDcLimMaxInt output; ActTq_Inp_mDragTq output AD_ActTq_tMDRAGTQ size=[1]; SplyU48_uU48 output; Tolerance constant single =0.01; CS_PrmM_fTqGrdSelect_XDB input; ElmTqLim_mTqMin output; CS_PrmM_nHSpdBd_XDF32 parameter; CS_PrmM_nLwrSpdBd_XDF32 parameter; TqMinInterpol local; CS_PrmM_uDcMaxVoltMode_XDF32 parameter; CS_PrmM_uDcMinVoltMode_XDF32 parameter
